simulink library "WECSim_Lib_Constraints"  (R2020b)
settings: Solver=VariableStepAuto  StartTime=0.0  StopTime=10.0  RelTol=1e-3
undefined symbols (not defined in the file or in its folder): constraint, simu, X, Y, Z
libraries: nesl_utility x48, sm_lib x34, WECSim_Lib_Body_Elements x1
(part 1 of 2)
settings Model: Creator=kmruehl  LastModifiedBy=akeeste

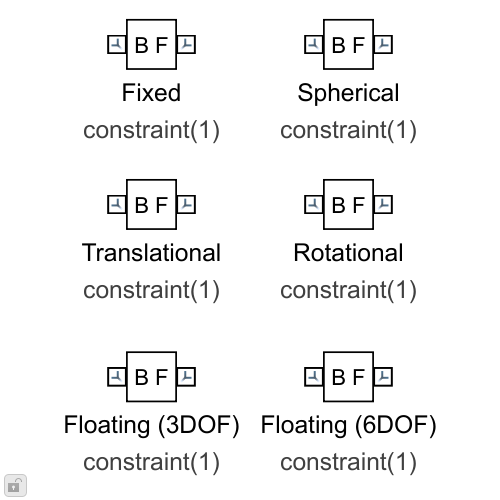
[thumbnail: Simulink's stored preview of the top-level diagram]
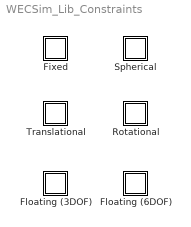
== system WECSim_Lib_Constraints ==
  Fixed : Subsystem  mask(Constraints){constraint=constraint(1)}
      mask prompts: constraint "Constraint Name:"
      mask help:
      | Constrains the follower to be fixed relative to the base.
      |
      | The variable name input below must be 'constraint(i)' where i=1,2,...
      | constraint(i) must be defined in the input file with the following fields:
      |
      |     .name (required)
      |             String.
      |             Constraint name. Must comply with Matlab's variable naming rules.
      |     .location (optional)
      |             3x1 vector [x y z] in meters.
      |             Constraint location. Default = [0 0 0]
      mask init:
      | if exist('constraint','var')
      |     h=[gcb '/To Workspace'];
      |     responseName=['constraint' num2str(constraint.number) '_out'];
      |     set_param(h,'VariableName',responseName);
      | end
      | 
      | constraint.checkLoc('W');
      settings: AttributesFormatString=%<constraint>
      mask Help:
      | Constrains the follower to be fixed relative to the base.
      | 
      | The variable name input below must be 'constraint(i)' where i=1,2,...
      | constraint(i) must be defined in the input file with the following fields:
      | 
      |     .name (required)
      |             String.
      |             Constraint name. Must comply with Matlab's variable naming rules.
      |     .location (optional)
      |             3x1 vector [x y z] in meters.
      |             Constraint location. Default = [0 0 0]
  Floating (3DOF) : Subsystem  mask(Constraints){constraint=constraint(1)}
      mask prompts: constraint "Constraint Name:"
      mask help:
      | Constraints the follower to planar motion relative to the base, linear
      | motions in the constraint's X- and Z- directions and rotational motion
      | about the constraint's Y-axis.
      |
      |
      | The variable name input below must be 'constraint(i)' where i=1,2,...
      | constraint(i) must be defined in the input file with the following fields:
      |
      |     .name (required)
      |             String.
      |             Constraint name. Must comply with Matlab's variable naming rules.
      |     .location (optional)
      |             3x1 vector [x y z] in meters.
      |             Constraint location. Default = [0 0 0]
      |     .orientation.z (optional)
      |             3x1 vector [x y z].
      |             Direction of the constraint's Z-coordinate. Default = [0 0 1]
      |     .orientation.y (optional)
      |             3x1 vector [x y z].
      |             Direction of the constraint's Y-coordinate. Default = [0 1 0]
      mask init: same as WECSim_Lib_Constraints/Fixed
      settings: AttributesFormatString=%<constraint>
      mask Help:
      | Constraints the follower to planar motion relative to the base, linear
      | motions in the constraint's X- and Z- directions and rotational motion
      | about the constraint's Y-axis.
      | 
      | 
      | The variable name input below must be 'constraint(i)' where i=1,2,...
      | constraint(i) must be defined in the input file with the following fields:
      | 
      |     .name (required)
      |             String.
      |             Constraint name. Must comply with Matlab's variable naming rules.
      |     .location (optional)
      |             3x1 vector [x y z] in meters.
      |             Constraint location. Default = [0 0 0]
      |     .orientation.z (optional)
      |             3x1 vector [x y z].
      |             Direction of the constraint's Z-coordinate. Default = [0 0 1]
      |     .orientation.y (optional)
      |             3x1 vector [x y z].
      |             Direction of the constraint's Y-coordinate. Default = [0 1 0]
  Floating (6DOF) : Subsystem  mask(Constraints){constraint=constraint(1)}
      mask prompts: constraint "Constraint Name:"
      mask help:
      | Allows unconstrained motion of the follower relative to the base in all 6
      | degrees of freedom.
      |
      |
      | The variable name input below must be 'constraint(i)' where i=1,2,...
      | constraint(i) must be defined in the input file with the following fields:
      |
      |     .name (required)
      |             String.
      |             Constraint name. Must comply with Matlab's variable naming rules.
      |     .location (optional)
      |             3x1 vector [x y z] in meters.
      |             Constraint location. Default = [0 0 0]
      |     .orientation.z (optional)
      |             3x1 vector [x y z].
      |             Direction of the constraint's Z-coordinate. Default = [0 0 1]
      |     .orientation.y (optional)
      |             3x1 vector [x y z].
      |             Direction of the constraint's Y-coordinate. Default = [0 1 0]
      mask init: same as WECSim_Lib_Constraints/Fixed
      settings: AttributesFormatString=%<constraint>
      mask Help:
      | Allows unconstrained motion of the follower relative to the base in all 6
      | degrees of freedom.
      | 
      | 
      | The variable name input below must be 'constraint(i)' where i=1,2,...
      | constraint(i) must be defined in the input file with the following fields:
      | 
      |     .name (required)
      |             String.
      |             Constraint name. Must comply with Matlab's variable naming rules.
      |     .location (optional)
      |             3x1 vector [x y z] in meters.
      |             Constraint location. Default = [0 0 0]
      |     .orientation.z (optional)
      |             3x1 vector [x y z].
      |             Direction of the constraint's Z-coordinate. Default = [0 0 1]
      |     .orientation.y (optional)
      |             3x1 vector [x y z].
      |             Direction of the constraint's Y-coordinate. Default = [0 1 0]
  Rotational : Subsystem  mask(Constraints){constraint=constraint(1)}
      mask prompts: constraint "Constraint Name:"
      mask help:
      | Constraints the follower to rotational motion relative to the base, about
      | the constraint's Y-axis. Location is required and affects dynamics.
      |
      |
      | The variable name input below must be 'constraint(i)' where i=1,2,...
      | constraint(i) must be defined in the input file with the following fields:
      |
      |     .name (required)
      |             String.
      |             Constraint name. Must comply with Matlab's variable naming rules.
      |     .location (required)
      |             3x1 vector [x y z] in meters.
      |             Constraint location. Default = [0 0 0]
      |     .orientation.z (optional)
      |             3x1 vector [x y z].
      |             Direction of the constraint's Z-coordinate. Default = [0 0 1]
      |     .orientation.y (optional)
      |             3x1 vector [x y z].
      |             Direction of the constraint's Y-coordinate. Default = [0 1 0]
      mask init:
      | if exist('constraint','var')
      |     h=[gcb '/To Workspace'];
      |     responseName=['constraint' num2str(constraint.number) '_out'];
      |     set_param(h,'VariableName',responseName);
      |     h=[gcb '/CONSTRAINT (Revolute Joint)'];
      |     try % this should catch any version issue for which these parameters do not exist
      |         set_param(h,'upperLimitSpecify',constraint.hardStops.upperLimitSpecify)
      |         set_param(h,'lowerLimitSpecify',constraint.hardStops.lowerLimitSpecify)
      |     end
      |     if constraint.extension.PositionTargetSpecify == 1
      |         set_param(h,'PositionTargetSpecify','on')
      |     else
      |         set_param(h,'PositionTargetSpecify','off')
      |     end
      | end
      | 
      | constraint.checkLoc('E');
      settings: AttributesFormatString=%<constraint>
      mask Help:
      | Constraints the follower to rotational motion relative to the base, about
      | the constraint's Y-axis. Location is required and affects dynamics.
      | 
      | 
      | The variable name input below must be 'constraint(i)' where i=1,2,...
      | constraint(i) must be defined in the input file with the following fields:
      | 
      |     .name (required)
      |             String.
      |             Constraint name. Must comply with Matlab's variable naming rules.
      |     .location (required)
      |             3x1 vector [x y z] in meters.
      |             Constraint location. Default = [0 0 0]
      |     .orientation.z (optional)
      |             3x1 vector [x y z].
      |             Direction of the constraint's Z-coordinate. Default = [0 0 1]
      |     .orientation.y (optional)
      |             3x1 vector [x y z].
      |             Direction of the constraint's Y-coordinate. Default = [0 1 0]
  Spherical : Subsystem  mask(Constraints){constraint=constraint(1)}
      mask prompts: constraint "Constraint Name:"
      mask help:
      | Constrains the follower to rotational motion relative to the base, fixing in
      | X,Y,Z but allowing rotation about each axis.
      |
      | The variable name input below must be 'constraint(i)' where i=1,2,...
      | constraint(i) must be defined in the input file with the following fields:
      |
      |     .name (required)
      |             String.
      |            Constraint name. Must comply with Matlab's variable naming rules.
      |     .location (optional)
      |             3x1 vector [x y z] in meters.
      |             Constraint location. Default = [0 0 0]
      |     .orientation.z (optional)
      |             3x1 vector [x y z].
      |             Direction of the constraint's Z-coordinate. Default = [0 0 1]
      |     .orientation.y (optional)
      |             3x1 vector [x y z].
      |             Direction of the constraint's Y-coordinate. Default = [0 1 0]
      mask init:
      | if exist('constraint','var')
      |     h=[gcb '/To Workspace'];
      |     responseName=['constraint' num2str(constraint.number) '_out'];
      |     set_param(h,'VariableName',responseName);
      |     h=[gcb '/Spherical Joint'];
      |     if constraint.extension.PositionTargetSpecify == 1
      |         set_param(h,'PositionTargetSpecify','on')
      |     else
      |         set_param(h,'PositionTargetSpecify','off')
      |     end
      | end
      | 
      | constraint.checkLoc('W');
      settings: AttributesFormatString=%<constraint>
      mask Help:
      | Constrains the follower to rotational motion relative to the base, fixing in
      | X,Y,Z but allowing rotation about each axis.
      | 
      | The variable name input below must be 'constraint(i)' where i=1,2,...
      | constraint(i) must be defined in the input file with the following fields:
      | 
      |     .name (required)
      |             String.
      |            Constraint name. Must comply with Matlab's variable naming rules.
      |     .location (optional)
      |             3x1 vector [x y z] in meters.
      |             Constraint location. Default = [0 0 0]
      |     .orientation.z (optional)
      |             3x1 vector [x y z].
      |             Direction of the constraint's Z-coordinate. Default = [0 0 1]
      |     .orientation.y (optional)
      |             3x1 vector [x y z].
      |             Direction of the constraint's Y-coordinate. Default = [0 1 0]
  Translational : Subsystem  mask(Constraints){constraint=constraint(1)}
      mask prompts: constraint "Constraint Name:"
      mask help:
      | Constraints the follower to translational motion relative to the base, in the constraint's Z-direction.
      |
      |
      | The variable name input below must be 'constraint(i)' where i=1,2,...
      | constraint(i) must be defined in the input file with the following fields:
      |
      |     .name (required)
      |             String.
      |             Constraint name. Must comply with Matlab's variable naming rules.
      |     .location (optional)
      |             3x1 vector [x y z] in meters.
      |             Constraint location. Default = [0 0 0]
      |     .orientation.z (optional)
      |             3x1 vector [x y z].
      |             Direction of the constraint's Z-coordinate. Default = [0 0 1]
      |     .orientation.y (optional)
      |             3x1 vector [x y z].
      |             Direction of the constraint's Y-coordinate. Default = [0 1 0]
      mask init:
      | if exist('constraint','var')
      |     h=[gcb '/To Workspace'];
      |     responseName=['constraint' num2str(constraint.number) '_out'];
      |     set_param(h,'VariableName',responseName);
      |     h=[gcb '/CONSTRAINT (Prismatic Joint)'];
      |     try % this should catch any version issue for which these parameters do not exist
      |         set_param(h,'upperLimitSpecify',constraint.hardStops.upperLimitSpecify)
      |         set_param(h,'lowerLimitSpecify',constraint.hardStops.lowerLimitSpecify)
      |     end
      |     if constraint.extension.PositionTargetSpecify == 1
      |         set_param(h,'PositionTargetSpecify','on')
      |     else
      |         set_param(h,'PositionTargetSpecify','off')
      |     end
      | end
      | constraint.checkLoc('W');
      settings: AttributesFormatString=%<constraint>
      mask Help:
      | Constraints the follower to translational motion relative to the base, in the constraint's Z-direction.
      | 
      | 
      | The variable name input below must be 'constraint(i)' where i=1,2,...
      | constraint(i) must be defined in the input file with the following fields:
      | 
      |     .name (required)
      |             String.
      |             Constraint name. Must comply with Matlab's variable naming rules.
      |     .location (optional)
      |             3x1 vector [x y z] in meters.
      |             Constraint location. Default = [0 0 0]
      |     .orientation.z (optional)
      |             3x1 vector [x y z].
      |             Direction of the constraint's Z-coordinate. Default = [0 0 1]
      |     .orientation.y (optional)
      |             3x1 vector [x y z].
      |             Direction of the constraint's Y-coordinate. Default = [0 1 0]

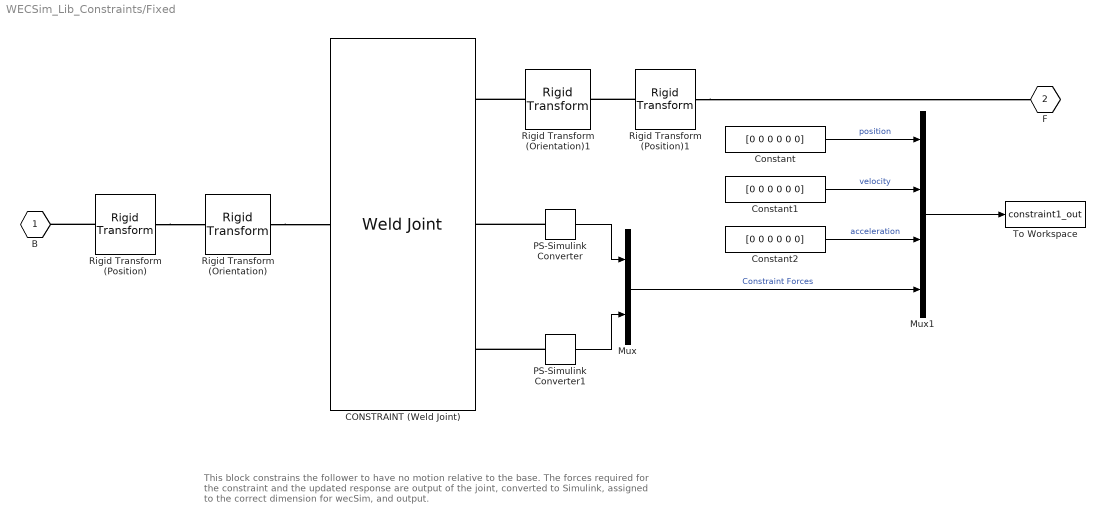
== system WECSim_Lib_Constraints/Fixed ==
  note: This block constrains the follower to have no motion relative to the base. The forces required for the constraint and the updated response are output of the joint, converted to Simulink, assigned to the correct dimension for wecSim, and output.
  CONSTRAINT (Weld Joint) : sm_lib/Joints/Weld Joint  JointMode=Normal  CompositeWrenchDir=BaseOnFollower  CompositeWrenchFrame=BaseFrame  SenseConstraintForce=on  SenseConstraintTorque=on  SenseTotalForce=off  SenseTotalTorque=off
  Constant : Constant  Value=[0 0 0 0 0 0]
  Constant1 : Constant  Value=[0 0 0 0 0 0]
  Constant2 : Constant  Value=[0 0 0 0 0 0]
  Mux : Mux  Inputs=2
  Mux1 : Mux
  PS-Simulink Converter : nesl_utility/PS-Simulink Converter  PhysicalDomain=network_engine_domain  SubClassName=ps_output  LeftPortType=input  RightPortType=output  PseudoPeriodic=off  Frequencies=[]  VectorFormat=1-D array  Unit=1  AffineConversion=off
  PS-Simulink Converter1 : nesl_utility/PS-Simulink Converter  PhysicalDomain=network_engine_domain  SubClassName=ps_output  LeftPortType=input  RightPortType=output  PseudoPeriodic=off  Frequencies=[]  VectorFormat=1-D array  Unit=1  AffineConversion=off
  Rigid Transform (Position) : sm_lib/Frames and Transforms/Rigid Transform  RotationMethod=None  FollAlignAxisA=+X  BaseAlignAxisA=+Y  FollAlignAxisB=+Y  BaseAlignAxisB=+Z  RotationStandardAxis=+Y  RotationAngle=0  RotationAngleUnits=rad  RotationArbitraryAxis=[0 1 0]  RotationSequenceAxes=FollowerAxes  RotationSequence=XYX  RotationSequenceAngles=[0 0 0]  RotationSequenceAnglesUnits=deg  RotationMatrix=[1 0 0; 0 1 0; 0 0 1]  Quaternion=[1 0 0 0]  TranslationMethod=Cartesian  TranslationCartesianOffset=constraint.initial.displacement+constraint.location  TranslationCartesianOffsetUnits=m  TranslationStandardAxis=+Z  TranslationStandardOffset=0  TranslationStandardOffsetUnits=m  TranslationROffset=0  TranslationROffsetUnits=m  TranslationThetaOffset=0  TranslationThetaOffsetUnits=deg  TranslationZOffset=0  TranslationZOffsetUnits=m
  Rigid Transform (Position)1 : sm_lib/Frames and Transforms/Rigid Transform  RotationMethod=None  FollAlignAxisA=+X  BaseAlignAxisA=+Y  FollAlignAxisB=+Y  BaseAlignAxisB=+Z  RotationStandardAxis=+Y  RotationAngle=0  RotationAngleUnits=rad  RotationArbitraryAxis=[0 1 0]  RotationSequenceAxes=FollowerAxes  RotationSequence=XYX  RotationSequenceAngles=[0 0 0]  RotationSequenceAnglesUnits=deg  RotationMatrix=[1 0 0; 0 1 0; 0 0 1]  Quaternion=[1 0 0 0]  TranslationMethod=Cartesian  TranslationCartesianOffset=constraint.initial.displacement+constraint.location  TranslationCartesianOffsetUnits=m  TranslationStandardAxis=+Z  TranslationStandardOffset=0  TranslationStandardOffsetUnits=m  TranslationROffset=0  TranslationROffsetUnits=m  TranslationThetaOffset=0  TranslationThetaOffsetUnits=deg  TranslationZOffset=0  TranslationZOffsetUnits=m
  Rigid Transform (Orientation) : sm_lib/Frames and Transforms/Rigid Transform  RotationMethod=RotationMatrix  FollAlignAxisA=+X  BaseAlignAxisA=+Y  FollAlignAxisB=+Y  BaseAlignAxisB=+Z  RotationStandardAxis=+Y  RotationAngle=0  RotationAngleUnits=rad  RotationArbitraryAxis=[0 1 0]  RotationSequenceAxes=FollowerAxes  RotationSequence=XYX  RotationSequenceAngles=[0 0 0]  RotationSequenceAnglesUnits=deg  RotationMatrix=constraint.orientation.rotationMatrix  Quaternion=[1 0 0 0]  TranslationMethod=None  TranslationCartesianOffset=constraint.location  TranslationCartesianOffsetUnits=m  TranslationStandardAxis=+Z  TranslationStandardOffset=0  TranslationStandardOffsetUnits=m  TranslationROffset=0  TranslationROffsetUnits=m  TranslationThetaOffset=0  TranslationThetaOffsetUnits=deg  TranslationZOffset=0  TranslationZOffsetUnits=m
  Rigid Transform (Orientation)1 : sm_lib/Frames and Transforms/Rigid Transform  RotationMethod=RotationMatrix  FollAlignAxisA=+X  BaseAlignAxisA=+Y  FollAlignAxisB=+Y  BaseAlignAxisB=+Z  RotationStandardAxis=+Y  RotationAngle=0  RotationAngleUnits=rad  RotationArbitraryAxis=[0 1 0]  RotationSequenceAxes=FollowerAxes  RotationSequence=XYX  RotationSequenceAngles=[0 0 0]  RotationSequenceAnglesUnits=deg  RotationMatrix=constraint.orientation.rotationMatrix  Quaternion=[1 0 0 0]  TranslationMethod=None  TranslationCartesianOffset=constraint.location  TranslationCartesianOffsetUnits=m  TranslationStandardAxis=+Z  TranslationStandardOffset=0  TranslationStandardOffsetUnits=m  TranslationROffset=0  TranslationROffsetUnits=m  TranslationThetaOffset=0  TranslationThetaOffsetUnits=deg  TranslationZOffset=0  TranslationZOffsetUnits=m
  To Workspace : ToWorkspace  VariableName=constraint1_out  SaveFormat=Structure With Time  SampleTime=simu.dtOut
  B : PMIOPort  Side=Left
  F : PMIOPort  Port=2  Side=Right
  wires:
  PS-Simulink Converter1/1 -> Mux/2
  PS-Simulink Converter/1 -> Mux/1
  Mux/1 -> Mux1/4  "Constraint Forces"
  Mux1/1 -> To Workspace/1
  Constant/1 -> Mux1/1  "position"
  Constant1/1 -> Mux1/2  "velocity"
  Constant2/1 -> Mux1/3  "acceleration"
  connections:
  Rigid Transform (Position)1/RConn1 -- Rigid Transform (Orientation)1/LConn1
  Rigid Transform (Position)/RConn1 -- Rigid Transform (Orientation)/LConn1
  Rigid Transform (Orientation)1/RConn1 -- CONSTRAINT (Weld Joint)/RConn1
  Rigid Transform (Position)1/LConn1 -- F/RConn1
  PS-Simulink Converter1/LConn1 -- CONSTRAINT (Weld Joint)/RConn3
  PS-Simulink Converter/LConn1 -- CONSTRAINT (Weld Joint)/RConn2
  Rigid Transform (Orientation)/RConn1 -- CONSTRAINT (Weld Joint)/LConn1
  Rigid Transform (Position)/LConn1 -- B/RConn1

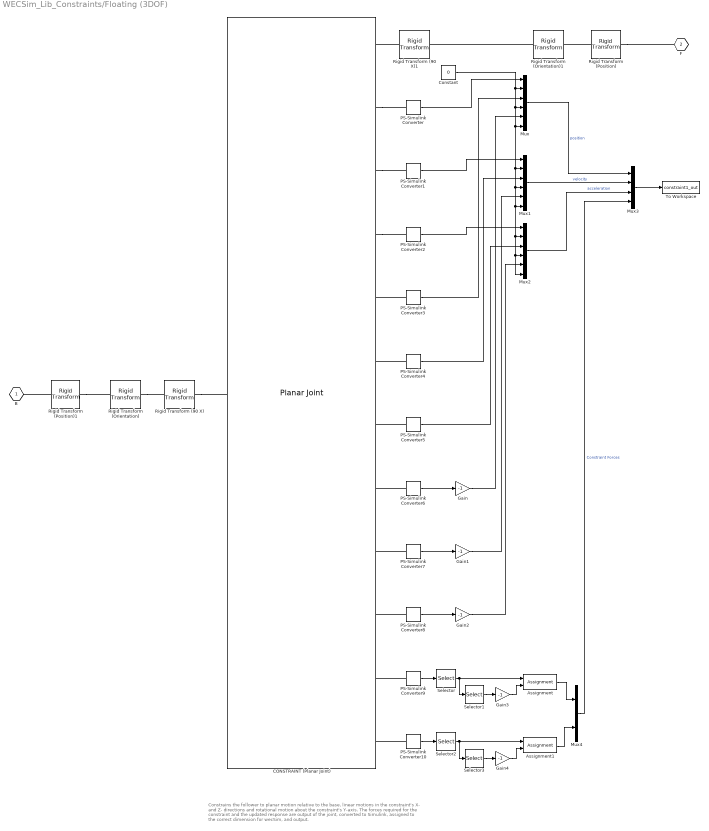
== system WECSim_Lib_Constraints/Floating (3DOF) ==
  note: Constrains the follower to planar motion relative to the base, linear
      | motions in the constraint's X- and Z- directions and rotational motion
      | about the constraint's Y-axis. The forces required for the constraint and the updated response are output of the joint, converted to Simulink, assigned to the correct dimension for wecSim, and output.
  Assignment : Assignment  DiagnosticForDimensions=Warning  IndexOptions=Index vector (dialog)  Indices=2  OutputSizes=1
  Assignment1 : Assignment  DiagnosticForDimensions=Warning  IndexOptions=Index vector (dialog)  Indices=2  OutputSizes=1
  CONSTRAINT (Planar Joint) : sm_lib/Joints/Planar Joint  JointMode=Normal  CompositeWrenchDir=BaseOnFollower  CompositeWrenchFrame=BaseFrame  SenseConstraintForce=on  SenseConstraintTorque=on  SenseTotalForce=off  SenseTotalTorque=off  PxPositionTargetSpecify=off  PxPositionTargetPriority=High  PxPositionTargetValue=0  PxPositionTargetValueUnits=m  PxVelocityTargetSpecify=off  PxVelocityTargetPriority=High  PxVelocityTargetValue=0  PxVelocityTargetValueUnits=m/s  PxEquilibriumPosition=0  PxEquilibriumPositionUnits=m  PxSpringStiffness=0  PxSpringStiffnessUnits=N/m  PxDampingCoefficient=0  PxDampingCoefficientUnits=N/(m/s)  PxLowerLimitSpecify=off  PxLowerLimitBound=-1  PxLowerLimitBoundUnits=m  PxLowerLimitStiffness=1e6  PxLowerLimitStiffnessUnits=N/m  PxLowerLimitDamping=1e3  PxLowerLimitDampingUnits=N/(m/s)  PxLowerLimitTransitionRegionWidth=1e-4  PxLowerLimitTransitionRegionWidthUnits=m  PxUpperLimitSpecify=off  PxUpperLimitBound=1  PxUpperLimitBoundUnits=m  PxUpperLimitStiffness=1e6  PxUpperLimitStiffnessUnits=N/m  PxUpperLimitDamping=1e3  PxUpperLimitDampingUnits=N/(m/s)  PxUpperLimitTransitionRegionWidth=1e-4  PxUpperLimitTransitionRegionWidthUnits=m  PxTorqueActuationMode=NoTorque  PxMotionActuationMode=ComputedMotion  PxSensePosition=on  PxSenseVelocity=on  PxSenseAcceleration=on  PxSenseTorqueForce=off  PxSenseLowerLimitTorqueForce=off  PxSenseUpperLimitTorqueForce=off  PyPositionTargetSpecify=off  PyPositionTargetPriority=High  PyPositionTargetValue=0  PyPositionTargetValueUnits=m  PyVelocityTargetSpecify=off  PyVelocityTargetPriority=High  PyVelocityTargetValue=0  PyVelocityTargetValueUnits=m/s  PyEquilibriumPosition=0  PyEquilibriumPositionUnits=m  PySpringStiffness=0  PySpringStiffnessUnits=N/m  PyDampingCoefficient=0  PyDampingCoefficientUnits=N/(m/s)  PyLowerLimitSpecify=off  PyLowerLimitBound=-1  PyLowerLimitBoundUnits=m  PyLowerLimitStiffness=1e6  PyLowerLimitStiffnessUnits=N/m  PyLowerLimitDamping=1e3  PyLowerLimitDampingUnits=N/(m/s)  PyLowerLimitTransitionRegionWidth=1e-4  PyLowerLimitTransitionRegionWidthUnits=m  PyUpperLimitSpecify=off  PyUpperLimitBound=1  PyUpperLimitBoundUnits=m  PyUpperLimitStiffness=1e6  PyUpperLimitStiffnessUnits=N/m  PyUpperLimitDamping=1e3  PyUpperLimitDampingUnits=N/(m/s)  PyUpperLimitTransitionRegionWidth=1e-4  PyUpperLimitTransitionRegionWidthUnits=m  PyTorqueActuationMode=NoTorque  PyMotionActuationMode=ComputedMotion  PySensePosition=on  PySenseVelocity=on  PySenseAcceleration=on  PySenseTorqueForce=off  PySenseLowerLimitTorqueForce=off  PySenseUpperLimitTorqueForce=off  RzPositionTargetSpecify=off  RzPositionTargetPriority=High  RzPositionTargetValue=0  RzPositionTargetValueUnits=deg  RzVelocityTargetSpecify=off  RzVelocityTargetPriority=High  RzVelocityTargetValue=0  RzVelocityTargetValueUnits=deg/s  RzEquilibriumPosition=0  RzEquilibriumPositionUnits=deg  RzSpringStiffness=0  RzSpringStiffnessUnits=N*m/deg  RzDampingCoefficient=0  RzDampingCoefficientUnits=N*m/(deg/s)  RzLowerLimitSpecify=off  RzLowerLimitBound=-90  RzLowerLimitBoundUnits=deg  RzLowerLimitStiffness=1e4  RzLowerLimitStiffnessUnits=N*m/deg  RzLowerLimitDamping=10  RzLowerLimitDampingUnits=N*m/(deg/s)  RzLowerLimitTransitionRegionWidth=0.1  RzLowerLimitTransitionRegionWidthUnits=deg  RzUpperLimitSpecify=off  RzUpperLimitBound=90  RzUpperLimitBoundUnits=deg  RzUpperLimitStiffness=1e4  RzUpperLimitStiffnessUnits=N*m/deg  RzUpperLimitDamping=10  RzUpperLimitDampingUnits=N*m/(deg/s)  RzUpperLimitTransitionRegionWidth=0.1  RzUpperLimitTransitionRegionWidthUnits=deg  RzTorqueActuationMode=NoTorque  RzMotionActuationMode=ComputedMotion  RzSensePosition=on  RzSenseVelocity=on  RzSenseAcceleration=on  RzSenseTorqueForce=off  RzSenseLowerLimitTorqueForce=off  RzSenseUpperLimitTorqueForce=off
  Constant : Constant  Value=0
  Gain{,1..4} (5 alike) : Gain  Gain=-1
  Mux : Mux  Inputs=6
  Mux1 : Mux  Inputs=6
  Mux2 : Mux  Inputs=6
  Mux3 : Mux
  Mux4 : Mux  Inputs=2
  PS-Simulink Converter{,1..10} (11 alike) : nesl_utility/PS-Simulink Converter  PhysicalDomain=network_engine_domain  SubClassName=ps_output  LeftPortType=input  RightPortType=output  PseudoPeriodic=off  Frequencies=[]  VectorFormat=1-D array  Unit=1  AffineConversion=off
  Rigid Transform (Position) : sm_lib/Frames and Transforms/Rigid Transform  RotationMethod=None  FollAlignAxisA=+X  BaseAlignAxisA=+Y  FollAlignAxisB=+Y  BaseAlignAxisB=+Z  RotationStandardAxis=+Y  RotationAngle=0  RotationAngleUnits=rad  RotationArbitraryAxis=[0 1 0]  RotationSequenceAxes=FollowerAxes  RotationSequence=XYX  RotationSequenceAngles=[0 0 0]  RotationSequenceAnglesUnits=deg  RotationMatrix=[1 0 0; 0 1 0; 0 0 1]  Quaternion=[1 0 0 0]  TranslationMethod=Cartesian  TranslationCartesianOffset=constraint.initial.displacement+constraint.location  TranslationCartesianOffsetUnits=m  TranslationStandardAxis=+Z  TranslationStandardOffset=0  TranslationStandardOffsetUnits=m  TranslationROffset=0  TranslationROffsetUnits=m  TranslationThetaOffset=0  TranslationThetaOffsetUnits=deg  TranslationZOffset=0  TranslationZOffsetUnits=m
  Rigid Transform (Position)1 : sm_lib/Frames and Transforms/Rigid Transform  RotationMethod=None  FollAlignAxisA=+X  BaseAlignAxisA=+Y  FollAlignAxisB=+Y  BaseAlignAxisB=+Z  RotationStandardAxis=+Y  RotationAngle=0  RotationAngleUnits=rad  RotationArbitraryAxis=[0 1 0]  RotationSequenceAxes=FollowerAxes  RotationSequence=XYX  RotationSequenceAngles=[0 0 0]  RotationSequenceAnglesUnits=deg  RotationMatrix=[1 0 0; 0 1 0; 0 0 1]  Quaternion=[1 0 0 0]  TranslationMethod=Cartesian  TranslationCartesianOffset=constraint.initial.displacement+constraint.location  TranslationCartesianOffsetUnits=m  TranslationStandardAxis=+Z  TranslationStandardOffset=0  TranslationStandardOffsetUnits=m  TranslationROffset=0  TranslationROffsetUnits=m  TranslationThetaOffset=0  TranslationThetaOffsetUnits=deg  TranslationZOffset=0  TranslationZOffsetUnits=m
  Rigid Transform (90 X) : sm_lib/Frames and Transforms/Rigid Transform  RotationMethod=StandardAxis  FollAlignAxisA=+X  BaseAlignAxisA=+Y  FollAlignAxisB=+Y  BaseAlignAxisB=+Z  RotationStandardAxis=+X  RotationAngle=90  RotationAngleUnits=deg  RotationArbitraryAxis=[0 1 0]  RotationSequenceAxes=FollowerAxes  RotationSequence=XYX  RotationSequenceAngles=[0 0 0]  RotationSequenceAnglesUnits=deg  RotationMatrix=[1 0 0; 0 1 0; 0 0 1]  Quaternion=[1 0 0 0]  TranslationMethod=None  TranslationCartesianOffset=constraint.location  TranslationCartesianOffsetUnits=m  TranslationStandardAxis=+Z  TranslationStandardOffset=0  TranslationStandardOffsetUnits=m  TranslationROffset=0  TranslationROffsetUnits=m  TranslationThetaOffset=0  TranslationThetaOffsetUnits=deg  TranslationZOffset=0  TranslationZOffsetUnits=m
  Rigid Transform (90 X)1 : sm_lib/Frames and Transforms/Rigid Transform  RotationMethod=StandardAxis  FollAlignAxisA=+X  BaseAlignAxisA=+Y  FollAlignAxisB=+Y  BaseAlignAxisB=+Z  RotationStandardAxis=+X  RotationAngle=90  RotationAngleUnits=deg  RotationArbitraryAxis=[0 1 0]  RotationSequenceAxes=FollowerAxes  RotationSequence=XYX  RotationSequenceAngles=[0 0 0]  RotationSequenceAnglesUnits=deg  RotationMatrix=[1 0 0; 0 1 0; 0 0 1]  Quaternion=[1 0 0 0]  TranslationMethod=None  TranslationCartesianOffset=constraint.location  TranslationCartesianOffsetUnits=m  TranslationStandardAxis=+Z  TranslationStandardOffset=0  TranslationStandardOffsetUnits=m  TranslationROffset=0  TranslationROffsetUnits=m  TranslationThetaOffset=0  TranslationThetaOffsetUnits=deg  TranslationZOffset=0  TranslationZOffsetUnits=m
  Rigid Transform (Orientation) : sm_lib/Frames and Transforms/Rigid Transform  RotationMethod=RotationMatrix  FollAlignAxisA=+X  BaseAlignAxisA=+Y  FollAlignAxisB=+Y  BaseAlignAxisB=+Z  RotationStandardAxis=+Y  RotationAngle=0  RotationAngleUnits=rad  RotationArbitraryAxis=[0 1 0]  RotationSequenceAxes=FollowerAxes  RotationSequence=XYX  RotationSequenceAngles=[0 0 0]  RotationSequenceAnglesUnits=deg  RotationMatrix=constraint.orientation.rotationMatrix  Quaternion=[1 0 0 0]  TranslationMethod=None  TranslationCartesianOffset=constraint.location  TranslationCartesianOffsetUnits=m  TranslationStandardAxis=+Z  TranslationStandardOffset=0  TranslationStandardOffsetUnits=m  TranslationROffset=0  TranslationROffsetUnits=m  TranslationThetaOffset=0  TranslationThetaOffsetUnits=deg  TranslationZOffset=0  TranslationZOffsetUnits=m
  Rigid Transform (Orientation)1 : sm_lib/Frames and Transforms/Rigid Transform  RotationMethod=RotationMatrix  FollAlignAxisA=+X  BaseAlignAxisA=+Y  FollAlignAxisB=+Y  BaseAlignAxisB=+Z  RotationStandardAxis=+Y  RotationAngle=0  RotationAngleUnits=rad  RotationArbitraryAxis=[0 1 0]  RotationSequenceAxes=FollowerAxes  RotationSequence=XYX  RotationSequenceAngles=[0 0 0]  RotationSequenceAnglesUnits=deg  RotationMatrix=constraint.orientation.rotationMatrix  Quaternion=[1 0 0 0]  TranslationMethod=None  TranslationCartesianOffset=constraint.location  TranslationCartesianOffsetUnits=m  TranslationStandardAxis=+Z  TranslationStandardOffset=0  TranslationStandardOffsetUnits=m  TranslationROffset=0  TranslationROffsetUnits=m  TranslationThetaOffset=0  TranslationThetaOffsetUnits=deg  TranslationZOffset=0  TranslationZOffsetUnits=m
  Selector : Selector  InputPortWidth=3  IndexOptions=Index vector (dialog)  Indices=[1 3 2]  OutputSizes=1
  Selector1 : Selector  InputPortWidth=3  IndexOptions=Index vector (dialog)  Indices=[2]  OutputSizes=1
  Selector2 : Selector  InputPortWidth=3  IndexOptions=Index vector (dialog)  Indices=[1 3 2]  OutputSizes=1
  Selector3 : Selector  InputPortWidth=3  IndexOptions=Index vector (dialog)  Indices=[2]  OutputSizes=1
  To Workspace : ToWorkspace  VariableName=constraint1_out  SaveFormat=Structure With Time  SampleTime=simu.dtOut
  B : PMIOPort  Side=Left
  F : PMIOPort  Port=2  Side=Right
  wires:
  Assignment/1 -> Mux4/1
  Assignment1/1 -> Mux4/2
  PS-Simulink Converter10/1 -> Selector2/1
  Gain4/1 -> Assignment1/2
  Selector3/1 -> Gain4/1
  Selector2/1 -> Assignment1/1, Selector3/1
  Constant/1 -> Mux/2, Mux1/2, Mux2/2, Mux2/6, Mux2/4, Mux1/6, Mux1/4, Mux/6, Mux/4
  Gain2/1 -> Mux2/5
  Gain1/1 -> Mux1/5
  Gain/1 -> Mux/5
  PS-Simulink Converter8/1 -> Gain2/1
  PS-Simulink Converter7/1 -> Gain1/1
  PS-Simulink Converter6/1 -> Gain/1
  PS-Simulink Converter5/1 -> Mux2/3
  PS-Simulink Converter4/1 -> Mux1/3
  PS-Simulink Converter3/1 -> Mux/3
  PS-Simulink Converter2/1 -> Mux2/1
  PS-Simulink Converter1/1 -> Mux1/1
  PS-Simulink Converter/1 -> Mux/1
  Gain3/1 -> Assignment/2
  Selector1/1 -> Gain3/1
  Selector/1 -> Selector1/1, Assignment/1
  PS-Simulink Converter9/1 -> Selector/1
  Mux4/1 -> Mux3/4  "Constraint Forces"
  Mux3/1 -> To Workspace/1
  Mux/1 -> Mux3/1  "position"
  Mux1/1 -> Mux3/2  "velocity"
  Mux2/1 -> Mux3/3  "acceleration"
  connections:
  Rigid Transform (Position)1/RConn1 -- Rigid Transform (Orientation)/LConn1
  Rigid Transform (Orientation)1/RConn1 -- Rigid Transform (90 X)1/LConn1
  Rigid Transform (Orientation)/RConn1 -- Rigid Transform (90 X)/LConn1
  Rigid Transform (Position)/RConn1 -- Rigid Transform (Orientation)1/LConn1
  Rigid Transform (90 X)/RConn1 -- CONSTRAINT (Planar Joint)/LConn1
  Rigid Transform (90 X)1/RConn1 -- CONSTRAINT (Planar Joint)/RConn1
  PS-Simulink Converter9/LConn1 -- CONSTRAINT (Planar Joint)/RConn11
  PS-Simulink Converter3/LConn1 -- CONSTRAINT (Planar Joint)/RConn5
  PS-Simulink Converter7/LConn1 -- CONSTRAINT (Planar Joint)/RConn9
  PS-Simulink Converter8/LConn1 -- CONSTRAINT (Planar Joint)/RConn10
  PS-Simulink Converter6/LConn1 -- CONSTRAINT (Planar Joint)/RConn8
  PS-Simulink Converter5/LConn1 -- CONSTRAINT (Planar Joint)/RConn7
  PS-Simulink Converter4/LConn1 -- CONSTRAINT (Planar Joint)/RConn6
  PS-Simulink Converter10/LConn1 -- CONSTRAINT (Planar Joint)/RConn12
  Rigid Transform (Position)/LConn1 -- F/RConn1
  Rigid Transform (Position)1/LConn1 -- B/RConn1
  CONSTRAINT (Planar Joint)/RConn2 -- PS-Simulink Converter/LConn1
  CONSTRAINT (Planar Joint)/RConn3 -- PS-Simulink Converter1/LConn1
  CONSTRAINT (Planar Joint)/RConn4 -- PS-Simulink Converter2/LConn1

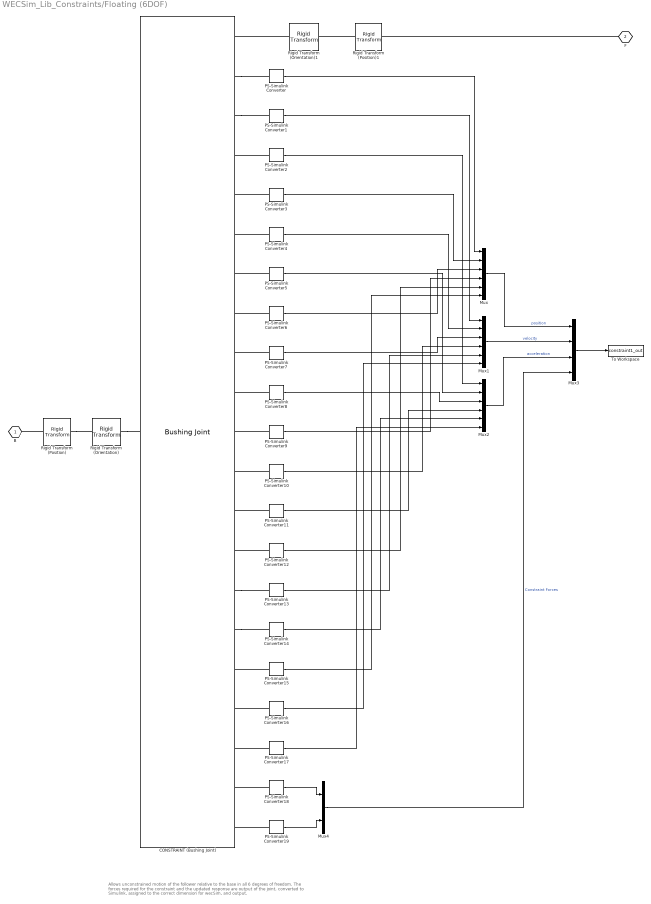
== system WECSim_Lib_Constraints/Floating (6DOF) ==
  note: Allows unconstrained motion of the follower relative to the base in all 6
      | degrees of freedom. The forces required for the constraint and the updated response are output of the joint, converted to Simulink, assigned to the correct dimension for wecSim, and output.
  CONSTRAINT (Bushing Joint) : sm_lib/Joints/Bushing Joint  JointMode=Normal  CompositeWrenchDir=BaseOnFollower  CompositeWrenchFrame=BaseFrame  SenseConstraintForce=on  SenseConstraintTorque=on  SenseTotalForce=off  SenseTotalTorque=off  PxPositionTargetSpecify=off  PxPositionTargetPriority=High  PxPositionTargetValue=0  PxPositionTargetValueUnits=m  PxVelocityTargetSpecify=off  PxVelocityTargetPriority=High  PxVelocityTargetValue=0  PxVelocityTargetValueUnits=m/s  PxEquilibriumPosition=0  PxEquilibriumPositionUnits=m  PxSpringStiffness=0  PxSpringStiffnessUnits=N/m  PxDampingCoefficient=0  PxDampingCoefficientUnits=N/(m/s)  PxLowerLimitSpecify=off  PxLowerLimitBound=-1  PxLowerLimitBoundUnits=m  PxLowerLimitStiffness=1e6  PxLowerLimitStiffnessUnits=N/m  PxLowerLimitDamping=1e3  PxLowerLimitDampingUnits=N/(m/s)  PxLowerLimitTransitionRegionWidth=1e-4  PxLowerLimitTransitionRegionWidthUnits=m  PxUpperLimitSpecify=off  PxUpperLimitBound=1  PxUpperLimitBoundUnits=m  PxUpperLimitStiffness=1e6  PxUpperLimitStiffnessUnits=N/m  PxUpperLimitDamping=1e3  PxUpperLimitDampingUnits=N/(m/s)  PxUpperLimitTransitionRegionWidth=1e-4  PxUpperLimitTransitionRegionWidthUnits=m  PxTorqueActuationMode=NoTorque  PxMotionActuationMode=ComputedMotion  PxSensePosition=on  PxSenseVelocity=on  PxSenseAcceleration=on  PxSenseTorqueForce=off  PxSenseLowerLimitTorqueForce=off  PxSenseUpperLimitTorqueForce=off  PyPositionTargetSpecify=off  PyPositionTargetPriority=High  PyPositionTargetValue=0  PyPositionTargetValueUnits=m  PyVelocityTargetSpecify=off  PyVelocityTargetPriority=High  PyVelocityTargetValue=0  PyVelocityTargetValueUnits=m/s  PyEquilibriumPosition=0  PyEquilibriumPositionUnits=m  PySpringStiffness=0  PySpringStiffnessUnits=N/m  PyDampingCoefficient=0  PyDampingCoefficientUnits=N/(m/s)  PyLowerLimitSpecify=off  PyLowerLimitBound=-1  PyLowerLimitBoundUnits=m  PyLowerLimitStiffness=1e6  PyLowerLimitStiffnessUnits=N/m  PyLowerLimitDamping=1e3  PyLowerLimitDampingUnits=N/(m/s)  PyLowerLimitTransitionRegionWidth=1e-4  PyLowerLimitTransitionRegionWidthUnits=m  PyUpperLimitSpecify=off  PyUpperLimitBound=1  PyUpperLimitBoundUnits=m  PyUpperLimitStiffness=1e6  PyUpperLimitStiffnessUnits=N/m  PyUpperLimitDamping=1e3  PyUpperLimitDampingUnits=N/(m/s)  PyUpperLimitTransitionRegionWidth=1e-4  PyUpperLimitTransitionRegionWidthUnits=m  PyTorqueActuationMode=NoTorque  PyMotionActuationMode=ComputedMotion  PySensePosition=on  PySenseVelocity=on  PySenseAcceleration=on  PySenseTorqueForce=off  PySenseLowerLimitTorqueForce=off  PySenseUpperLimitTorqueForce=off  PzPositionTargetSpecify=off  PzPositionTargetPriority=High  PzPositionTargetValue=0  PzPositionTargetValueUnits=m  PzVelocityTargetSpecify=off  PzVelocityTargetPriority=High  PzVelocityTargetValue=0  PzVelocityTargetValueUnits=m/s  PzEquilibriumPosition=0  PzEquilibriumPositionUnits=m  PzSpringStiffness=0  PzSpringStiffnessUnits=N/m  PzDampingCoefficient=0  PzDampingCoefficientUnits=N/(m/s)  PzLowerLimitSpecify=off  PzLowerLimitBound=-1  PzLowerLimitBoundUnits=m  PzLowerLimitStiffness=1e6  PzLowerLimitStiffnessUnits=N/m  PzLowerLimitDamping=1e3  PzLowerLimitDampingUnits=N/(m/s)  PzLowerLimitTransitionRegionWidth=1e-4  PzLowerLimitTransitionRegionWidthUnits=m  PzUpperLimitSpecify=off  PzUpperLimitBound=1  PzUpperLimitBoundUnits=m  PzUpperLimitStiffness=1e6  PzUpperLimitStiffnessUnits=N/m  PzUpperLimitDamping=1e3  PzUpperLimitDampingUnits=N/(m/s)  PzUpperLimitTransitionRegionWidth=1e-4  PzUpperLimitTransitionRegionWidthUnits=m  PzTorqueActuationMode=NoTorque  PzMotionActuationMode=ComputedMotion  PzSensePosition=on  PzSenseVelocity=on  PzSenseAcceleration=on  PzSenseTorqueForce=off  PzSenseLowerLimitTorqueForce=off  PzSenseUpperLimitTorqueForce=off  RxPositionTargetSpecify=off  RxPositionTargetPriority=High  RxPositionTargetValue=0  RxPositionTargetValueUnits=deg  RxVelocityTargetSpecify=off  RxVelocityTargetPriority=High  RxVelocityTargetValue=0  RxVelocityTargetValueUnits=deg/s  RxEquilibriumPosition=0  RxEquilibriumPositionUnits=deg  RxSpringStiffness=0  RxSpringStiffnessUnits=N*m/deg  RxDampingCoefficient=0  RxDampingCoefficientUnits=N*m/(deg/s)  RxLowerLimitSpecify=off  RxLowerLimitBound=-90  RxLowerLimitBoundUnits=deg  RxLowerLimitStiffness=1e4  RxLowerLimitStiffnessUnits=N*m/deg  RxLowerLimitDamping=10  RxLowerLimitDampingUnits=N*m/(deg/s)  RxLowerLimitTransitionRegionWidth=0.1  RxLowerLimitTransitionRegionWidthUnits=deg  RxUpperLimitSpecify=off  RxUpperLimitBound=90  RxUpperLimitBoundUnits=deg  RxUpperLimitStiffness=1e4  RxUpperLimitStiffnessUnits=N*m/deg  RxUpperLimitDamping=10  RxUpperLimitDampingUnits=N*m/(deg/s)  RxUpperLimitTransitionRegionWidth=0.1  RxUpperLimitTransitionRegionWidthUnits=deg  RxTorqueActuationMode=NoTorque  RxMotionActuationMode=ComputedMotion  RxSensePosition=on  RxSenseVelocity=on  RxSenseAcceleration=on  RxSenseTorqueForce=off  RxSenseLowerLimitTorqueForce=off  RxSenseUpperLimitTorqueForce=off  RyPositionTargetSpecify=off  RyPositionTargetPriority=High  RyPositionTargetValue=0  RyPositionTargetValueUnits=deg  RyVelocityTargetSpecify=off  RyVelocityTargetPriority=High  RyVelocityTargetValue=0  RyVelocityTargetValueUnits=deg/s  RyEquilibriumPosition=0  RyEquilibriumPositionUnits=deg  RySpringStiffness=0  RySpringStiffnessUnits=N*m/deg  RyDampingCoefficient=0  RyDampingCoefficientUnits=N*m/(deg/s)  RyLowerLimitSpecify=off  RyLowerLimitBound=-90  RyLowerLimitBoundUnits=deg  RyLowerLimitStiffness=1e4  RyLowerLimitStiffnessUnits=N*m/deg  RyLowerLimitDamping=10  RyLowerLimitDampingUnits=N*m/(deg/s)  RyLowerLimitTransitionRegionWidth=0.1  RyLowerLimitTransitionRegionWidthUnits=deg  RyUpperLimitSpecify=off  RyUpperLimitBound=90  RyUpperLimitBoundUnits=deg  RyUpperLimitStiffness=1e4  RyUpperLimitStiffnessUnits=N*m/deg  RyUpperLimitDamping=10  RyUpperLimitDampingUnits=N*m/(deg/s)  RyUpperLimitTransitionRegionWidth=0.1  RyUpperLimitTransitionRegionWidthUnits=deg  RyTorqueActuationMode=NoTorque  RyMotionActuationMode=ComputedMotion  RySensePosition=on  RySenseVelocity=on  RySenseAcceleration=on  RySenseTorqueForce=off  RySenseLowerLimitTorqueForce=off  RySenseUpperLimitTorqueForce=off  RzPositionTargetSpecify=off  RzPositionTargetPriority=High  RzPositionTargetValue=0  RzPositionTargetValueUnits=deg  RzVelocityTargetSpecify=off  RzVelocityTargetPriority=High  RzVelocityTargetValue=0  RzVelocityTargetValueUnits=deg/s  RzEquilibriumPosition=0  RzEquilibriumPositionUnits=deg  RzSpringStiffness=0  RzSpringStiffnessUnits=N*m/deg  RzDampingCoefficient=0  RzDampingCoefficientUnits=N*m/(deg/s)  RzLowerLimitSpecify=off  RzLowerLimitBound=-90  RzLowerLimitBoundUnits=deg  RzLowerLimitStiffness=1e4  RzLowerLimitStiffnessUnits=N*m/deg  RzLowerLimitDamping=10  RzLowerLimitDampingUnits=N*m/(deg/s)  RzLowerLimitTransitionRegionWidth=0.1  RzLowerLimitTransitionRegionWidthUnits=deg  RzUpperLimitSpecify=off  RzUpperLimitBound=90  RzUpperLimitBoundUnits=deg  RzUpperLimitStiffness=1e4  RzUpperLimitStiffnessUnits=N*m/deg  RzUpperLimitDamping=10  RzUpperLimitDampingUnits=N*m/(deg/s)  RzUpperLimitTransitionRegionWidth=0.1  RzUpperLimitTransitionRegionWidthUnits=deg  RzTorqueActuationMode=NoTorque  RzMotionActuationMode=ComputedMotion  RzSensePosition=on  RzSenseVelocity=on  RzSenseAcceleration=on  RzSenseTorqueForce=off  RzSenseLowerLimitTorqueForce=off  RzSenseUpperLimitTorqueForce=off
  Mux : Mux  Inputs=6
  Mux1 : Mux  Inputs=6
  Mux2 : Mux  Inputs=6
  Mux3 : Mux
  Mux4 : Mux  Inputs=2
  PS-Simulink Converter{,1..19} (20 alike) : nesl_utility/PS-Simulink Converter  PhysicalDomain=network_engine_domain  SubClassName=ps_output  LeftPortType=input  RightPortType=output  PseudoPeriodic=off  Frequencies=[]  VectorFormat=1-D array  Unit=1  AffineConversion=off
  Rigid Transform (Position) : sm_lib/Frames and Transforms/Rigid Transform  RotationMethod=None  FollAlignAxisA=+X  BaseAlignAxisA=+Y  FollAlignAxisB=+Y  BaseAlignAxisB=+Z  RotationStandardAxis=+Y  RotationAngle=0  RotationAngleUnits=rad  RotationArbitraryAxis=[0 1 0]  RotationSequenceAxes=FollowerAxes  RotationSequence=XYX  RotationSequenceAngles=[0 0 0]  RotationSequenceAnglesUnits=deg  RotationMatrix=[1 0 0; 0 1 0; 0 0 1]  Quaternion=[1 0 0 0]  TranslationMethod=Cartesian  TranslationCartesianOffset=constraint.initial.displacement+constraint.location  TranslationCartesianOffsetUnits=m  TranslationStandardAxis=+Z  TranslationStandardOffset=0  TranslationStandardOffsetUnits=m  TranslationROffset=0  TranslationROffsetUnits=m  TranslationThetaOffset=0  TranslationThetaOffsetUnits=deg  TranslationZOffset=0  TranslationZOffsetUnits=m
  Rigid Transform (Position)1 : sm_lib/Frames and Transforms/Rigid Transform  RotationMethod=None  FollAlignAxisA=+X  BaseAlignAxisA=+Y  FollAlignAxisB=+Y  BaseAlignAxisB=+Z  RotationStandardAxis=+Y  RotationAngle=0  RotationAngleUnits=rad  RotationArbitraryAxis=[0 1 0]  RotationSequenceAxes=FollowerAxes  RotationSequence=XYX  RotationSequenceAngles=[0 0 0]  RotationSequenceAnglesUnits=deg  RotationMatrix=[1 0 0; 0 1 0; 0 0 1]  Quaternion=[1 0 0 0]  TranslationMethod=Cartesian  TranslationCartesianOffset=constraint.initial.displacement+constraint.location  TranslationCartesianOffsetUnits=m  TranslationStandardAxis=+Z  TranslationStandardOffset=0  TranslationStandardOffsetUnits=m  TranslationROffset=0  TranslationROffsetUnits=m  TranslationThetaOffset=0  TranslationThetaOffsetUnits=deg  TranslationZOffset=0  TranslationZOffsetUnits=m
  Rigid Transform (Orientation) : sm_lib/Frames and Transforms/Rigid Transform  RotationMethod=RotationMatrix  FollAlignAxisA=+X  BaseAlignAxisA=+Y  FollAlignAxisB=+Y  BaseAlignAxisB=+Z  RotationStandardAxis=+Y  RotationAngle=0  RotationAngleUnits=rad  RotationArbitraryAxis=[0 1 0]  RotationSequenceAxes=FollowerAxes  RotationSequence=XYX  RotationSequenceAngles=[0 0 0]  RotationSequenceAnglesUnits=deg  RotationMatrix=constraint.orientation.rotationMatrix  Quaternion=[1 0 0 0]  TranslationMethod=None  TranslationCartesianOffset=constraint.location  TranslationCartesianOffsetUnits=m  TranslationStandardAxis=+Z  TranslationStandardOffset=0  TranslationStandardOffsetUnits=m  TranslationROffset=0  TranslationROffsetUnits=m  TranslationThetaOffset=0  TranslationThetaOffsetUnits=deg  TranslationZOffset=0  TranslationZOffsetUnits=m
  Rigid Transform (Orientation)1 : sm_lib/Frames and Transforms/Rigid Transform  RotationMethod=RotationMatrix  FollAlignAxisA=+X  BaseAlignAxisA=+Y  FollAlignAxisB=+Y  BaseAlignAxisB=+Z  RotationStandardAxis=+Y  RotationAngle=0  RotationAngleUnits=rad  RotationArbitraryAxis=[0 1 0]  RotationSequenceAxes=FollowerAxes  RotationSequence=XYX  RotationSequenceAngles=[0 0 0]  RotationSequenceAnglesUnits=deg  RotationMatrix=constraint.orientation.rotationMatrix  Quaternion=[1 0 0 0]  TranslationMethod=None  TranslationCartesianOffset=constraint.location  TranslationCartesianOffsetUnits=m  TranslationStandardAxis=+Z  TranslationStandardOffset=0  TranslationStandardOffsetUnits=m  TranslationROffset=0  TranslationROffsetUnits=m  TranslationThetaOffset=0  TranslationThetaOffsetUnits=deg  TranslationZOffset=0  TranslationZOffsetUnits=m
  To Workspace : ToWorkspace  VariableName=constraint1_out  SaveFormat=Structure With Time  SampleTime=simu.dtOut
  B : PMIOPort  Side=Left
  F : PMIOPort  Port=2  Side=Right
  wires:
  PS-Simulink Converter17/1 -> Mux2/6
  PS-Simulink Converter16/1 -> Mux1/6
  PS-Simulink Converter15/1 -> Mux/6
  PS-Simulink Converter14/1 -> Mux2/5
  PS-Simulink Converter13/1 -> Mux1/5
  PS-Simulink Converter12/1 -> Mux/5
  PS-Simulink Converter11/1 -> Mux2/4
  PS-Simulink Converter10/1 -> Mux1/4
  PS-Simulink Converter9/1 -> Mux/4
  PS-Simulink Converter8/1 -> Mux2/3
  PS-Simulink Converter7/1 -> Mux1/3
  PS-Simulink Converter6/1 -> Mux/3
  PS-Simulink Converter5/1 -> Mux2/2
  PS-Simulink Converter4/1 -> Mux1/2
  PS-Simulink Converter3/1 -> Mux/2
  PS-Simulink Converter2/1 -> Mux2/1
  PS-Simulink Converter1/1 -> Mux1/1
  PS-Simulink Converter/1 -> Mux/1
  PS-Simulink Converter18/1 -> Mux4/1
  PS-Simulink Converter19/1 -> Mux4/2
  Mux4/1 -> Mux3/4  "Constraint Forces"
  Mux3/1 -> To Workspace/1
  Mux/1 -> Mux3/1  "position"
  Mux1/1 -> Mux3/2  "velocity"
  Mux2/1 -> Mux3/3  "acceleration"
  connections:
  Rigid Transform (Position)/RConn1 -- Rigid Transform (Orientation)/LConn1
  Rigid Transform (Position)1/RConn1 -- Rigid Transform (Orientation)1/LConn1
  Rigid Transform (Orientation)1/RConn1 -- CONSTRAINT (Bushing Joint)/RConn1
  Rigid Transform (Orientation)/RConn1 -- CONSTRAINT (Bushing Joint)/LConn1
  PS-Simulink Converter19/LConn1 -- CONSTRAINT (Bushing Joint)/RConn21
  PS-Simulink Converter18/LConn1 -- CONSTRAINT (Bushing Joint)/RConn20
  PS-Simulink Converter17/LConn1 -- CONSTRAINT (Bushing Joint)/RConn19
  PS-Simulink Converter16/LConn1 -- CONSTRAINT (Bushing Joint)/RConn18
  PS-Simulink Converter15/LConn1 -- CONSTRAINT (Bushing Joint)/RConn17
  CONSTRAINT (Bushing Joint)/RConn16 -- PS-Simulink Converter14/LConn1
  CONSTRAINT (Bushing Joint)/RConn15 -- PS-Simulink Converter13/LConn1
  PS-Simulink Converter12/LConn1 -- CONSTRAINT (Bushing Joint)/RConn14
  PS-Simulink Converter11/LConn1 -- CONSTRAINT (Bushing Joint)/RConn13
  PS-Simulink Converter10/LConn1 -- CONSTRAINT (Bushing Joint)/RConn12
  PS-Simulink Converter9/LConn1 -- CONSTRAINT (Bushing Joint)/RConn11
  PS-Simulink Converter8/LConn1 -- CONSTRAINT (Bushing Joint)/RConn10
  PS-Simulink Converter7/LConn1 -- CONSTRAINT (Bushing Joint)/RConn9
  PS-Simulink Converter6/LConn1 -- CONSTRAINT (Bushing Joint)/RConn8
  PS-Simulink Converter5/LConn1 -- CONSTRAINT (Bushing Joint)/RConn7
  PS-Simulink Converter4/LConn1 -- CONSTRAINT (Bushing Joint)/RConn6
  PS-Simulink Converter3/LConn1 -- CONSTRAINT (Bushing Joint)/RConn5
  PS-Simulink Converter2/LConn1 -- CONSTRAINT (Bushing Joint)/RConn4
  CONSTRAINT (Bushing Joint)/RConn3 -- PS-Simulink Converter1/LConn1
  CONSTRAINT (Bushing Joint)/RConn2 -- PS-Simulink Converter/LConn1
  Rigid Transform (Position)/LConn1 -- B/RConn1
  F/RConn1 -- Rigid Transform (Position)1/LConn1
